simulink model "Simulink_Rubrica_Cadena_Completa"  (R2023a)
settings: Solver=ode45  StartTime=0.0  StopTime=2.5  MaxStep=0.01  RelTol=1e-3
PreLoadFcn:
  | if ~exist('fis','var'), fis = readfis('ControlDifusoMotorDC.fis'); end
InitFcn:
  | if ~exist('fis','var'), fis = readfis('ControlDifusoMotorDC.fis'); end
libraries: fuzblock x1
settings Model: Creator=juanj  LastModifiedBy=juanj
settings RTWCC: GPUComputeCapability=5.0
settings ConfigComp: CovBoundaryAbsTol=1.0e-5

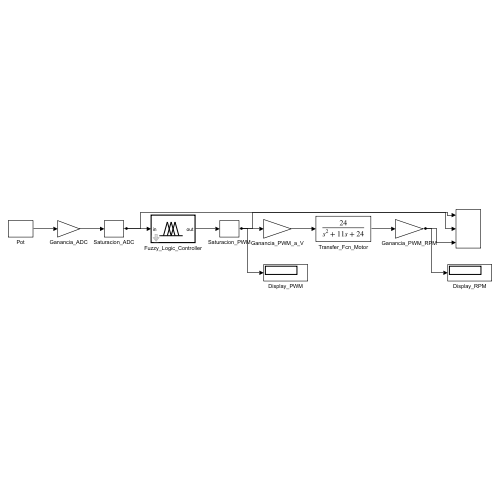
[thumbnail: Simulink's stored preview of the top-level diagram]
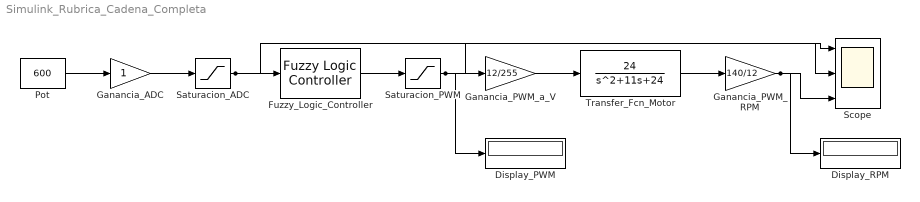
== system Simulink_Rubrica_Cadena_Completa ==
  Display_PWM : Display
  Display_RPM : Display
  Fuzzy_Logic_Controller : fuzblock/Fuzzy Logic  Controller  FIS=fis  OutputSampleNumber=101  DataType=double  FuzzifiedInputs=off  RuleFiringStrengths=off  RuleOutputs=off  AggregatedOutputs=off  SimulateUsing=Interpreted execution  OutOfRangeInputValueMessage=warning  NoRuleFiredMessage=warning  EmptyOutputFuzzySetMessage=warning
  Ganancia_ADC : Gain
  Ganancia_PWM_RPM : Gain  Gain=140/12
  Ganancia_PWM_a_V : Gain  Gain=12/255
  Pot : Constant  Value=600
  Saturacion_ADC : Saturate  UpperLimit=1023  LowerLimit=0
  Saturacion_PWM : Saturate  UpperLimit=255  LowerLimit=0
  Scope : Scope  NumInputPorts=3
  Transfer_Fcn_Motor : TransferFcn  Numerator=[24]  Denominator=[1 11 24]
  wires:
  Pot/1 -> Ganancia_ADC/1
  Ganancia_ADC/1 -> Saturacion_ADC/1
  Saturacion_ADC/1 -> Fuzzy_Logic_Controller/1, Scope/1
  Fuzzy_Logic_Controller/1 -> Saturacion_PWM/1
  Saturacion_PWM/1 -> Display_PWM/1, Ganancia_PWM_a_V/1, Scope/2
  Ganancia_PWM_a_V/1 -> Transfer_Fcn_Motor/1
  Transfer_Fcn_Motor/1 -> Ganancia_PWM_RPM/1
  Ganancia_PWM_RPM/1 -> Display_RPM/1, Scope/3
